simulink model "turbo_controller"  (R2025a)
settings: Solver=FixedStepAuto  StartTime=0.0  StopTime=inf  FixedStep=0.001  RelTol=1e-3
PostLoadFcn:
  | % 自动定位同目录CubeMX文件；不需要外部初始化脚本。
  | codertarget.data.setParameterValue('turbo_controller','STM32CubeMX.ProjectFile',fullfile(fileparts(get_param('turbo_controller','FileName')),'turbo_f407.ioc'));
InitFcn:
  | % 中文说明：按原控制器字段与类型创建三组接口总线；控制参数已内嵌。
  | tc_names=["EValve_Cycle" "EValve_Open" "Eblast_Cycle" "Eblast_Open" "Motor_Cycle" "Motor_Open" "EValve_Enable" "Eblast_Enable" "Motor_Enable" "SWO_Firework" "SWO_BleedAir" "EngineState" "Flag_ECUReset_Clear" "Flag_ECUReset_Save" "Flag_Reset_Enable" "Accelerator" "Nc_dem" "Nc"]; tc_types=["uint16" "uint16" "uint16" "uint16" "uint16" "uint16" "uint8" "uint8" "uint8" "uint8" "uint8" "uint8" "uint8" "uint8" "uint8" "single" "single" "single"];
  | for tc_k=1:numel(tc_names)
  |  tc_e(tc_k)=Simulink.BusElement; tc_e(tc_k).Name=char(tc_names(tc_k)); tc_e(tc_k).DataType=char(tc_types(tc_k));
  | end
  | EngineControl_Out=Simulink.Bus; EngineControl_Out.DataScope='Exported'; EngineControl_Out.Elements=tc_e;
  | clear tc_e tc_names tc_types tc_k
  | tc_names=["savedata1" "savedata2" "savedata3" "savedata4" "savedata5" "savedata6" "savedata7" "savedata8" "savedata9" "savedata10" "savedata11" "savedata12" "savedata13" "savedata14" "savedata15" "savedata16" "savedata17" "savedata18" "savedata19" "savedata20" "savedata21" "savedata22" "savedata23" "savedata24" "savedata25"]; tc_types=["single" "single" "single" "single" "single" "single" "single" "single" "single" "single" "single" "single" "single" "single" "single" "single" "single" "single" "single" "single" "single" "single" "single" "single" "single"];
  | for tc_k=1:numel(tc_names)
  |  tc_e(tc_k)=Simulink.BusElement; tc_e(tc_k).Name=char(tc_names(tc_k)); tc_e(tc_k).DataType=char(tc_types(tc_k));
  | end
  | SaveData_Out=Simulink.Bus; SaveData_Out.DataScope='Exported'; SaveData_Out.Elements=tc_e;
  | clear tc_e tc_names tc_types tc_k
  | tc_names=["senddata1" "senddata2" "senddata3" "senddata4" "senddata5" "senddata6" "senddata7" "senddata8" "senddata9" "senddata10" "senddata11" "senddata12" "senddata13" "senddata14" "senddata15" "senddata16" "senddata17" "senddata18" "senddata19" "senddata20" "senddata21" "senddata22" "senddata23" "senddata24" "senddata25" "senddata26" "senddata27" "senddata28" "senddata29"]; tc_types=["uint8" "uint8" "uint8" "uint8" "uint8" "uint8" "uint8" "uint8" "uint8" "uint8" "uint8" "uint8" "uint8" "uint8" "uint8" "uint8" "uint8" "uint8" "uint8" "uint8" "uint8" "uint8" "uint8" "uint8" "uint8" "uint8" "uint8" "uint8" "uint8"];
  | for tc_k=1:numel(tc_names)
  |  tc_e(tc_k)=Simulink.BusElement; tc_e(tc_k).Name=char(tc_names(tc_k)); tc_e(tc_k).DataType=char(tc_types(tc_k));
  | end
  | SendData_Out=Simulink.Bus; SendData_Out.DataScope='Exported'; SendData_Out.Elements=tc_e;
  | clear tc_e tc_names tc_types tc_k
  | 
  | % 以下为接口中文说明；只设置描述，不改变数值或数据类型。
  | EngineControl_Out.Description='执行控制输出（阀、电机、点火、状态及复位请求）';
  | tc_cn=["EValve_Cycle（主油阀周期计数（每计数2毫秒））" "EValve_Open（主油阀开通计数（每计数2毫秒））" "Eblast_Cycle（副油阀周期计数（每计数2毫秒））" "Eblast_Open（副油阀开通计数（每计数2毫秒））" "Motor_Cycle（起动电机周期计数）" "Motor_Open（起动电机开通计数）" "EValve_Enable（主油阀驱动使能）" "Eblast_Enable（副油阀驱动使能）" "Motor_Enable（起动电机使能）" "SWO_Firework（点火器使能（1开））" "SWO_BleedAir（引气阀使能（1开））" "EngineState（发动机状态）" "Flag_ECUReset_Clear（清除复位恢复状态请求）" "Flag_ECUReset_Save（保存复位恢复数据请求）" "Flag_Reset_Enable（处理器软件复位请求）" "Accelerator（油门／油泵给定控制量）" "Nc_dem（控制目标转速）" "Nc（发动机反馈转速（转每分））"];
  | tc_elements=EngineControl_Out.Elements;
  | for tc_k=1:numel(tc_cn)
  |  tc_elements(tc_k).Description=char(tc_cn(tc_k));
  | end
  | EngineControl_Out.Elements=tc_elements;
  | clear tc_cn tc_elements tc_k
  | SaveData_Out.Description='25项运行记录；字段含义按当前模型数据来源解释';
  | tc_cn=["savedata1（指令回显记录）" "savedata2（入口总温记录（℃））" "savedata3（电源电压记录）" "savedata4（排气温度记录（℃））" "savedata5（标定燃油压力记录）" "savedata6（副油阀占空比记录（％））" "savedata7（主油阀占空比记录（％））" "savedata8（温度修正转速记录）" "savedata9（开关输出及反馈位域）" "savedata10（物理转速记录）" "savedata11（油泵目标给定原始值）" "savedata12（起动电机占空比记录（％））" "savedata13（发动机状态码记录）" "savedata14（故障告警位域记录）" "savedata15（模型记录帧序号）" "savedata16（处理器温度记录（℃））" "savedata17（装订转速记录（沿用旧电源字段名））" "savedata18（导航高度记录）" "savedata19（飞行空速记录）" "savedata20（主阀旧记录位（恒零保留））" "savedata21（第21项保留记录（恒零））" "savedata22（保留记录项22）" "savedata23（保留记录项23）" "savedata24（保留记录项24）" "savedata25（保留记录项25）"];
  | tc_elements=SaveData_Out.Elements;
  | for tc_k=1:numel(tc_cn)
  |  tc_elements(tc_k).Description=char(tc_cn(tc_k));
  | end
  | SaveData_Out.Elements=tc_elements;
  | clear tc_cn tc_elements tc_k
  | SendData_Out.Description='29字段回传及外设命令接口；板端上位机帧只取第3至27字段';
  | tc_cn=["senddata1（回传发送允许标志（不直接上线路））" "senddata2（回传载荷长度25字节）" "senddata3（回传指令回显字节）" "senddata4（总温编码字节（℃＋80））" "senddata5（电源电压编码字节）" "senddata6（排温编码高字节）" "senddata7（排温编码低字节）" "senddata8（燃油压力编码高字节）" "senddata9（燃油压力编码低字节）" "senddata10（副油阀占空比字节（％））" "senddata11（主油阀占空比字节（％））" "senddata12（修正转速编码高字节）" "senddata13（修正转速编码低字节）" "senddata14（驱动及反馈状态位域）" "senddata15（物理转速编码高字节）" "senddata16（物理转速编码低字节）" "senddata17（油泵目标给定高字节（串口二使用））" "senddata18（油泵目标给定低字节（串口二使用））" "senddata19（起动电机占空比命令（串口一使用））" "senddata20（发动机状态码字节）" "senddata21（故障告警位域字节）" "senddata22（帧序号占位（板端另行填写））" "senddata23（处理器温度编码（℃＋50））" "senddata24（控制目标转速编码高字节）" "senddata25（控制目标转速编码低字节）" "senddata26（占位字节（板端改填实测泵速高字节））" "senddata27（占位字节（板端改填实测泵速低字节））" "senddata28（装订转速高字节（本板未发送））" "senddata29（装订转速低字节（本板未发送））"];
  | tc_elements=SendData_Out.Elements;
  | for tc_k=1:numel(tc_cn)
  |  tc_elements(tc_k).Description=char(tc_cn(tc_k));
  | end
  | SendData_Out.Elements=tc_elements;
  | clear tc_cn tc_elements tc_k
  | 
  | 
  | % FRAM模块化事务：接口类型和上电初始状态，随模型保存，无外部初始化文件。
  | clear FM_elements
  | FM_elements(1)=Simulink.BusElement;FM_elements(1).Name='phase';FM_elements(1).DataType='uint8';FM_elements(1).Dimensions=[1 1];FM_elements(1).Description='phase（当前事务阶段）';
  | FM_elements(2)=Simulink.BusElement;FM_elements(2).Name='a';FM_elements(2).DataType='uint8';FM_elements(2).Dimensions=[64 1];FM_elements(2).Description='a（启动时缓存的首区64字节）';
  | FM_elements(3)=Simulink.BusElement;FM_elements(3).Name='active';FM_elements(3).DataType='uint16';FM_elements(3).Dimensions=[1 1];FM_elements(3).Description='active（当前有效记录区地址）';
  | FM_elements(4)=Simulink.BusElement;FM_elements(4).Name='generation';FM_elements(4).DataType='uint32';FM_elements(4).Dimensions=[1 1];FM_elements(4).Description='generation（当前有效记录代号）';
  | FM_elements(5)=Simulink.BusElement;FM_elements(5).Name='record';FM_elements(5).DataType='uint8';FM_elements(5).Dimensions=[64 1];FM_elements(5).Description='record（本次冻结的待写记录）';
  | FM_elements(6)=Simulink.BusElement;FM_elements(6).Name='addr';FM_elements(6).DataType='uint16';FM_elements(6).Dimensions=[1 1];FM_elements(6).Description='addr（本次备用写入地址）';
  | FM_elements(7)=Simulink.BusElement;FM_elements(7).Name='lastSave';FM_elements(7).DataType='single';FM_elements(7).Dimensions=[1 1];FM_elements(7).Description='lastSave（上次开始保存的秒数）';
  | FM_elements(8)=Simulink.BusElement;FM_elements(8).Name='lastState';FM_elements(8).DataType='uint8';FM_elements(8).Dimensions=[1 1];FM_elements(8).Description='lastState（上次保存时的发动机状态）';
  | FM_elements(9)=Simulink.BusElement;FM_elements(9).Name='boot';FM_elements(9).DataType='boolean';FM_elements(9).Dimensions=[1 1];FM_elements(9).Description='boot（启动记录是否允许恢复）';
  | FM_elements(10)=Simulink.BusElement;FM_elements(10).Name='consumed';FM_elements(10).DataType='boolean';FM_elements(10).Dimensions=[1 1];FM_elements(10).Description='consumed（本次启动恢复通知是否已发送）';
  | FM_elements(11)=Simulink.BusElement;FM_elements(11).Name='payload';FM_elements(11).DataType='uint8';FM_elements(11).Dimensions=[20 1];FM_elements(11).Description='payload（当前20字节恢复内容）';
  | ... (+35 lines)
model workspace (MAT data in the model file):
  CRC16_Table_Reference = [0 4129 8258 12387 16516 20645 24774 28903 33032 37161 41290 45419 ... (256 elements, 256x1)]
  PE_Kaer = [0.15402 0.15402 0.12264 0.10076 0.09481 0.07601 0.07111 0.0569 0.05198 0.04926 0.05308 0.04325 ... (13 elements, 1x13)]
  PE_Nr = [21.2982 61.4260372 67.7475458 72.7394382 76.845934 80.6988798 83.8449282 86.6491912 88.9382406 89.178606 91.1938214 93.4068058 ... (13 elements, 1x13)]
  PE_Pump_Translate = 33.5999984741
  PE_RotaSpeed_Translate = 860
  PE_Taer = [0.4939154 0.4939154 0.40780982 0.34066978 0.31622756 0.30405716 0.34300244 0.26785022 0.37393554 0.23914836 0.44563948 0.31044662 ... (13 elements, 1x13)]
  PF_ACCFULLRANGE = 3360
  PF_Flag_ECUReset = 0
  PF_Flag_rx_suc = 1
  PF_Gear_Info = [40000; 45000; 50000; 55000; 57000; 59000; 60000; 61000; 61000; 61000; 61000; 61000]
  PF_K_TiaoJie = 1
  PF_Kpu = 10
  PF_MySet_Rxdata = [0 0 0 0 0 0 0 0 0 0 0 0 ... (50 elements, 50x1)]
  PF_MyUsart1_Rxdata = [0 0 0 0 0 0 0 0 0 0 0 0 ... (50 elements, 50x1)]
  PF_MyUsart2_Rxdata = [0 0 0 0 0 0 0 0 0 0 0 0 ... (50 elements, 50x1)]
  PF_Reset_Information = [0 0 0 0 0 0 0 0 0 0 0 0 ... (20 elements, 20x1)]
  PF_Sensor_X1_T4 = [0 4095]
  PF_Sensor_X2_T4 = [0 1.66666698456]
  PF_Sensor_X3_T4 = [0 504 999 1497 2010 2529 3051 3568 4076 4571 4959]
  PF_Sensor_X_P2 = [0.5 3]
  PF_Sensor_X_Poil = [0.5 3]
  PF_Sensor_X_T1t = [-50 300]
  PF_Sensor_X_Vpower = [0 3]
  PF_Sensor_X_Vpump = [0 3]
  PF_Sensor_Y1_T4 = [0 3]
  PF_Sensor_Y2_T4 = [0 5000]
  PF_Sensor_Y3_T4 = [0 100 200 300 400 500 600 700 800 900 980]
  PF_Sensor_Y_P2 = [0 1000]
  PF_Sensor_Y_Poil = [0 1000]
  PF_Sensor_Y_T1t = [-50 300]
  PF_Sensor_Y_Vpower = [0 33]
  PF_Sensor_Y_Vpump = [0 33]
  PG_CtrlMode_CloseLoop : mpt.Parameter (value not decoded)
  PG_CtrlMode_ManualAcc : mpt.Parameter (value not decoded)
  PG_CtrlMode_Origin : mpt.Parameter (value not decoded)
  PG_CtrlMode_Start : mpt.Parameter (value not decoded)
  PG_CtrlMode_Stop : mpt.Parameter (value not decoded)
  PG_ES_Clp : mpt.Parameter (value not decoded)
  PG_ES_EngStart : mpt.Parameter (value not decoded)
  PG_ES_Manual : mpt.Parameter (value not decoded)
  PG_ES_Origin : mpt.Parameter (value not decoded)
  PG_ES_Stop : mpt.Parameter (value not decoded)
  PG_Instr_BleedAirSet : mpt.Parameter (value not decoded)
  PG_Instr_CloseLoop : mpt.Parameter (value not decoded)
  PG_Instr_ECUReSet : mpt.Parameter (value not decoded)
  PG_Instr_EValveSet : mpt.Parameter (value not decoded)
  PG_Instr_EblastSet : mpt.Parameter (value not decoded)
  PG_Instr_Erase : mpt.Parameter (value not decoded)
  PG_Instr_FireWorkSet : mpt.Parameter (value not decoded)
  PG_Instr_ManualPlus : mpt.Parameter (value not decoded)
  PG_Instr_ManualrReduce : mpt.Parameter (value not decoded)
  PG_Instr_MotorSet : mpt.Parameter (value not decoded)
  PG_Instr_OilSet : mpt.Parameter (value not decoded)
  PG_Instr_SelfCheck : mpt.Parameter (value not decoded)
  PG_Instr_Start : mpt.Parameter (value not decoded)
  PG_Instr_Stop : mpt.Parameter (value not decoded)
  PG_Instr_StopZero : Simulink.Parameter (value not decoded)
  PG_Location_Air : Simulink.Parameter (value not decoded)
  PG_Location_Gnd : Simulink.Parameter (value not decoded)
  PG_ServoCtrlMode_CloseLoop : Simulink.Parameter (value not decoded)
  PG_ServoCtrlMode_CloseLoopMax : Simulink.Parameter (value not decoded)
  PG_ServoCtrlMode_CloseLoopMin : Simulink.Parameter (value not decoded)
  PG_ServoCtrlMode_ManualAcc : Simulink.Parameter (value not decoded)
  PG_ServoCtrlMode_ManualAccMax : Simulink.Parameter (value not decoded)
  PG_ServoCtrlMode_ManualAccMin : Simulink.Parameter (value not decoded)
  PG_SpeedDot_Permit : Simulink.Parameter (value not decoded)
  PL_EngineModel_Actuator = [0 10 100]
  PL_EngineModel_EngineStar_Press_P2 = [1013 1098.4 1099.144828 1099.931034 1103.613793 1162.662069 1143.793103 1131.006897 1123.186207 1117.6 1114 1111.806897 ... (127 elements, 1x127)]
  PL_EngineModel_EngineStar_RotaSpeed = [200 2000 9584 9660 10220 10240 10260 10288 10308 10368 10380 10408 ... (127 elements, 1x127)]
  PL_EngineModel_EngineStar_Temp_Exhaust = [128 129 129.1 130 131 131.1 132 133 134 134.1 135 135.1 ... (127 elements, 1x127)]
  PL_EngineModel_EngineStar_Time = [0.05 0.1 0.15 0.2 0.25 0.3 0.35 0.4 0.45 0.5 0.55 0.6 ... (127 elements, 1x127)]
  PL_EngineModel_IdleAbove_Nr = [0 21.2982 61.4260372 67.7475458 72.7394382 76.845934 80.6988798 83.8449282 86.6491912 88.9382406 89.178606 91.1938214 ... (14 elements, 1x14)]
  PL_EngineModel_IdleAbove_P2r = [0.986923266716 1.57907722675 1.81593881076 1.99358499877 2.23044658278 2.43770046879 2.65482358747 2.84233900814 3.03972366149 3.18776215149 3.25684678016 3.3950160375 ... (14 elements, 1x14)]
  PL_EngineModel_IdleAbove_Tempr = [0.0536001429337 1.07200285867 1.63301768805 1.63659103091 1.66875111667 1.72592460247 1.77595140254 1.86171163123 1.95461854565 2.03323208862 2.03323208862 2.13685903162 ... (14 elements, 1x14)]
  PL_EngineModel_IdleAbove_Ter = [0.42434128 0.42434128 0.42434128 0.30669408 0.23570008 0.22150128 0.1997974 0.23803274 0.16115638 0.24279948 0.13600422 0.31308354 ... (14 elements, 1x14)]
  PL_EngineModel_IdleAbove_Wfr = [0 10.142 23.8337 27.8905 31.9473 36.0041 40.0609 44.1177 48.1745 52.2313 52.7384 56.7952 ... (14 elements, 1x14)]
  PL_EngineModel_Press_P2 = [400 400 400 400 400 400 400 400 400 400]
  PL_EngineModel_Rotaspeed = [0 20000 96400]
  PL_EngineModel_Temp_Exhaust = [500 500 500 500 500 500 500 500 500 500]
  PL_Kaer = [0.1 0.1 0.1 0.1 0.1 0.1]
  PL_Nr = [50 60 70 80 90 100]
  PL_Taer = [0.1 0.1 0.1 0.1 0.1 0.1]
  Sig : Simulink.Signal (value not decoded)
  Ts_ms : Simulink.Parameter (value not decoded)
  false : Simulink.Parameter (value not decoded)
  true : Simulink.Parameter (value not decoded)
symbols that are objects in the model workspace (value not decoded): PG_CtrlMode_CloseLoop, PG_CtrlMode_ManualAcc, PG_CtrlMode_Origin, PG_CtrlMode_Start, PG_CtrlMode_Stop, PG_ES_Clp, PG_ES_EngStart, PG_ES_Manual, PG_ES_Origin, PG_ES_Stop, PG_Instr_BleedAirSet, PG_Instr_CloseLoop, PG_Instr_EblastSet, PG_Instr_ECUReSet, PG_Instr_Erase, PG_Instr_EValveSet, PG_Instr_FireWorkSet, PG_Instr_ManualPlus, PG_Instr_ManualrReduce, PG_Instr_MotorSet, PG_Instr_OilSet, PG_Instr_SelfCheck, PG_Instr_Start, PG_Instr_Stop, PG_Instr_StopZero, PG_ServoCtrlMode_CloseLoop, PG_ServoCtrlMode_CloseLoopMax, PG_ServoCtrlMode_CloseLoopMin, PG_ServoCtrlMode_ManualAcc, PG_ServoCtrlMode_ManualAccMax, PG_ServoCtrlMode_ManualAccMin, Ts_ms
libraries: simulink x97, stm32blockslib x10, stm32f4xxblockslib x8
(part 9 of 26)

== system turbo_controller/CLM/Start ==
  note: 普通起动：先记住起动前状态，再按阶段控制供油与电机
      |
      | 进入Start分支时，先保持起动前排温、油压；当前真正送入起动图的是油压参考，排温参考输出接终
      | 止端。参数支路根据滤波油压及历史参数准备初始电机开度、供油曲线和时间参数。
      |
      | Start_OpenLoop随后按A～F推进：准备、拖转、建立油压与供油、继续加速、退出起动电机、转入闭环
      | 。各阶段会同时修改油泵给定、主副油阀、电机和点火许可，并检查转速、油压与超时。
      |
      | 本系统只保留普通起动。阶段完成或异常的标志送回发动机状态管理，驱动量则经过统一输出管理后执
      | 行；内部某个阶段标志不是硬件执行成功的回执。
  note: DaYu5000
      | DaYu5000：只判断一个条件
      |
      | 把输入与5000比较，使用关系“>=”。成立输出1，不成立输出0；输出是判断标志，不是把输入缩放成
      | 该常数。
      |
      | 比较门限用于父级的分支条件，没有滤波、延时确认或锁存。例如输入恰好等于门限时，“>=、<=、==
      | ”成立，“>、<”不成立。是否需要持续确认或同时满足其他条件，由父级连线决定。
  S_SPM : Inport
      settings: AttributesFormatString=S_SPM（通信及传感器信息总线）
  S_ServoOut_Last : Inport  Port=2
      settings: AttributesFormatString=S_ServoOut_Last（伺服输出上一周期）
  S_Origin_T4 : Inport  Port=3
      settings: AttributesFormatString=S_Origin_T4（起动前保存的排温初值）
  S_Origin_POil : Inport  Port=4
      settings: AttributesFormatString=S_Origin_POil（起动前保存的燃油压力初值）
  Action Port : ActionPort  InitializeStates=reset  ActionPortLabel=case [ 1 ]:
      settings: AttributesFormatString=Action Port（动作端口）
  Bus Creator : BusCreator  Inputs=14
      settings: AttributesFormatString=Bus Creator（总线创建器）
  Bus Selector : BusSelector  OutputSignals=Sensor（传感器信息总线）.T4_Filter（滤波后排气温度）,Sensor（传感器信息总线）.Nc_Filter（滤波后转速）,Sensor（传感器信息总线）.POil_Filter（滤波后燃油压力）
      settings: AttributesFormatString=Bus Selector（总线选择器）
  Bus Selector2 : BusSelector  OutputSignals=m1（中间变量一）,m2（中间变量二）,m3（中间变量三）,m4（中间变量四）,n1（中间变量五）,n2（中间变量六）
      settings: AttributesFormatString=Bus Selector2（总线选择器2）
  Bus Selector3 : BusSelector  OutputSignals=m1（中间变量一）,m2（中间变量二）,m3（中间变量三）,m4（中间变量四）,n1（中间变量五）,n2（中间变量六）
      settings: AttributesFormatString=Bus Selector3（总线选择器3）
  Constant5 : Constant  Value=5000  OutDataTypeStr=single
      settings: AttributesFormatString=Constant5（常量5）
  Constant6 : Constant  Value=0  OutDataTypeStr=single
      settings: AttributesFormatString=Constant6（常量6）
  DaYu5000 : simulink/Logic and Bit Operations/Compare To Constant  Description=|  relop=>=  const=5000  OutDataTypeStr=boolean
      | DaYu5000：只判断一个条件
      | 
      | 把输入与5000比较，使用关系“>=”。成立输出1，不成立输出0；输出是判断标志，不是把输入缩放成该常数。
      | 
      | 比较门限用于父级的分支条件，没有滤波、延时确认或锁存。例如输入恰好等于门限时，“>=、<=、==”成立，“>、<”不成立。是否需要持续确认或同时满足其他条件，由父级连线决定。
      settings: AttributesFormatString=DaYu5000（大于五千）
  HoldFirst : Subsystem  Description=|
      | 保存进入起动时的排温和油压参考
      | 
      | 起动前的T4、油压会在进入本分支时被锁住。Hold图提供首次运行标志，外面的开关和延迟负责保存对应的传感器数值；不是Hold图自己保存两路模拟量。
      | 
      | 起动期间，即便当前排温或油压改变，参考值也保持进入时的水平。后面的起动图用“当前油压-起动前油压”判断压力是否建立。排温参考输出当前接Unused_OriginT4终止端，并未送入起动图；图内T4_01则在到达1000 rpm阶段另取当时排温。不能因为这里保持了两路，就认为两路都被采用。
      settings: AttributesFormatString=HoldFirst（保持首次）
  PG_CtrlMode_Start : Constant  Value=PG_CtrlMode_Start  OutDataTypeStr=uint8  SampleTime=-1
      settings: AttributesFormatString=PG_CtrlMode_Start（起动）
  PG_CtrlMode_Start3 : Constant  RequirementInfo={} %GIDa_444c69f1_f02a_4ad8_a0e8_71029ce8eb11  Value=Ts_ms  SampleTime=-1
      settings: AttributesFormatString=PG_CtrlMode_Start3（起动3）
  Range : Stateflow chart  Description=|  TreatAsAtomicUnit=on
      | 本实例把普通起动图产生的Accelerator限制在0～5000，输出为起动泵控制编码。图内算出的曲线即使大于5000也会在此截住。
      | 
      | 把一个数限制在允许范围内
      | 
      | 输入包括待处理值、允许下限和允许上限。先比较是否越过上限，越过就输出上限；未超过上限时再检查下限，小于下限就输出下限；落在范围内则原样通过。恰好等于边界的值也保留。
      | 
      | 计算式：输出 = min(max(输入，下限)，上限)。
      | 例如下限为0、上限为100时，输入120输出100，输入-5输出0，输入60输出60。这里不做平均、不计算变化速度，也不记住上一拍；它只防止当前数值越界。具体边界由父子系统连入，不能把此处的输出一律理解为百分比。
      settings: AttributesFormatString=Range（限幅或范围）
  Signal Conversion : SignalConversion  OverrideOpt=off
      settings: AttributesFormatString=Signal Conversion（信号转换）
  StartFault_Default : Constant  Description=原图该输出从未赋值，保持初始 false；显式常量保留现有起动总线字段。  Value=false  OutDataTypeStr=boolean
  Start_OpenLoop : Stateflow chart  Description=|  TreatAsAtomicUnit=on  RTWFcnName=Timmer  RTWFileName=MCM_Timmer
      | 普通起动的六阶段顺序控制
      | 
      | A准备：等待约1 s，记录并限制起动前油压参考，设置阀门周期、开启主副油路及电机使能。
      | B拖转：转速达到1000后进入C，开启点火并给出起动供油；约6 s仍未达到要求时走异常退出。
      | C建立油路：经过约3 s、油压相对基准上升50或已有进入标志时，调整主油阀与泵给定；按t、T参数和转速条件逐渐提高电机开通，达到100进入D。
      | D继续加速：转速超过参数n1进入E；超过约6 s未满足条件时撤销点火、清供油并设置异常阶段码。
      | E按转速供油：泵给定在(n1,m1)、(n2,m2)间按直线计算；超过13000时撤销起动电机和点火，超过20000进入F。油压持续高于700或本阶段约30 s超时也有退出分支。
      | F转闭环：转速超过28000或达到约20 s时关闭副油路；再按1 s、3 s的延迟恢复主油路和m4给定，最后申请进入闭环。
      | 
      | 转速单位rpm，T4为温度，油压阈值采用标定后的工程编码。计时统一按毫秒/Ts_ms比较；Ts_ms=20 ms时，1000 ms对应50次调用。泵曲线公式：
      | 泵给定=m1+(m2-m1)×(当前转速-n1)/(n2-n1)。
      | 
      | 这些阶段是流程标志，不是额外的AirStart或BWStart模式。电机关闭还有高转速及锁存路径，最终输出仍受父级模式和使能控制。
      settings: AttributesFormatString=Start_OpenLoop（地面起动开环时序）  RTWFcnNameOpts=Use subsystem name  RTWFileNameOpts=User specified
  Subsystem : Subsystem  Description=|
      | 为普通起动准备压力相关参数
      | 
      | 输入P来自POil_Filter（滤波燃油压力），不是环境静压或入口总压；另有和上一组供油曲线参数。初始化/计时支路控制何时继续沿用旧参数、何时采用压力查表结果，并由首次标志保存本次起动所需的初始值。
      | 
      | 滤波燃油压力按50～100的断点插值：初始电机开通NPump0由30变化到50，电机上升时间T由10变化到8，等待参数t由10变化到5。低压、高压会得到不同的起动节奏，不是直接把压力当作油泵开度。
      | 
      | 另一分支生成m1～m4和n1、n2供油曲线参数，再打成总线交给Start_OpenLoop。参数的含义是“在什么转速给多少泵编码、等待多久”，不代表实际油压已达到目标。
      settings: AttributesFormatString=Subsystem（子系统）
  Switch : Switch  Criteria=u2 ~= 0  SaturateOnIntegerOverflow=off  InputSameDT=off
      settings: AttributesFormatString=Switch（开关选择）
  Time Delay1 : UnitDelay  SampleTime=-1  HasFrameUpgradeWarning=on
      settings: AttributesFormatString=Time Delay1（时间延迟1）
  Unused_OriginT4 : Terminator
  Unused_ServoHistory : Terminator
  dth = T0-288.1 : Constant  Value=0  OutDataTypeStr=uint8  SampleTime=-1
      settings: AttributesFormatString=dth = T0-288.1（固定常量0（旧名称不参与计算））
  dth = T0-288.6 : Constant  OutDataTypeStr=uint8  SampleTime=-1
      settings: AttributesFormatString=dth = T0-288.6（固定常量1（旧名称不参与计算））
  S_CtrlMode_Start : Outport  InitialOutput=[0]
      settings: AttributesFormatString=S_CtrlMode_Start（控制模式起动）
  S_Start : Outport  Port=2
      settings: AttributesFormatString=S_Start（地面起动）
  wires:
  PG_CtrlMode_Start/1 -> S_CtrlMode_Start/1
  S_SPM/1 -> Bus Selector/1
  Start_OpenLoop/1(Accelerator) -> Range/1(In)
  Bus Creator/1 -> Signal Conversion/1
  Signal Conversion/1 -> S_Start/1
  Bus Selector/2 -> DaYu5000/1, Start_OpenLoop/2(Nc)  "<Nc_Filter（滤波后转速）>"
  Start_OpenLoop/7(Motor_Open) -> Bus Creator/7  "Motor_Open（起动电机开通计数）"
  Start_OpenLoop/6(Motor_Cycle) -> Bus Creator/6  "Motor_Cycle（起动电机周期计数）"
  Start_OpenLoop/8(EValve_Enable) -> Bus Creator/8  "EValve_Enable（主油阀使能）"
  Start_OpenLoop/5(Eblast_Open) -> Bus Creator/5  "Eblast_Open（副油阀开通计数）"
  Start_OpenLoop/9(Eblast_Enable) -> Bus Creator/9  "Eblast_Enable（副油阀使能）"
  Start_OpenLoop/4(Eblast_Cycle) -> Bus Creator/4  "Eblast_Cycle（副油阀周期计数）"
  Start_OpenLoop/10(Motor_Enable) -> Bus Creator/10  "Motor_Enable（起动电机使能）"
  Start_OpenLoop/3(EValve_Open) -> Bus Creator/3  "EValve_Open（主油阀开通计数）"
  Start_OpenLoop/11(SWO_Firework) -> Bus Creator/11  "SWO_Firework（点火器使能）"
  Start_OpenLoop/2(EValve_Cycle) -> Bus Creator/2  "EValve_Cycle（主油阀周期计数）"
  Start_OpenLoop/12(Flag_EngineState) -> Bus Creator/12  "Flag_RunState（运行状态标志）"
  S_Origin_T4/1 -> HoldFirst/1(S_Origin_T4)
  Switch/1 -> Bus Creator/14  "SWO_BleedAir（引气阀使能）"
  Bus Selector/1 -> Start_OpenLoop/1(T4)  "<T4_Filter（滤波后排气温度）>"
  PG_CtrlMode_Start3/1 -> Start_OpenLoop/13(Ts_ms)
  S_Origin_POil/1 -> HoldFirst/2(S_Origin_POil)
  HoldFirst/2(S_Origin_POil_1) -> Start_OpenLoop/14(Origin_POil)
  Bus Selector/3 -> Subsystem/1(P), Start_OpenLoop/3(POil)  "<POil_Filter（滤波后燃油压力）>"
  Constant6/1 -> Range/3(Min)
  Constant5/1 -> Range/2(Max)
  Range/1(Out) -> Bus Creator/1  "Start_Accelerator（地面起动油泵给定）"
  Time Delay1/1 -> Bus Selector2/1
  Bus Selector2/1 -> Subsystem/2(m1_last)  "<m1（中间变量一）>"
  Bus Selector2/2 -> Subsystem/3(m2_last)  "<m2（中间变量二）>"
  Bus Selector2/3 -> Subsystem/4(m3_last)  "<m3（中间变量三）>"
  Bus Selector2/4 -> Subsystem/5(m4_last)  "<m4（中间变量四）>"
  Subsystem/2(m) -> Time Delay1/1, Bus Selector3/1
  Bus Selector3/1 -> Start_OpenLoop/5(m1)  "<m1（中间变量一）>"
  Bus Selector3/2 -> Start_OpenLoop/6(m2)  "<m2（中间变量二）>"
  Bus Selector3/3 -> Start_OpenLoop/7(m3)  "<m3（中间变量三）>"
  Bus Selector3/4 -> Start_OpenLoop/8(m4)  "<m4（中间变量四）>"
  Subsystem/1(NPump0) -> Start_OpenLoop/4(NPump0)
  Subsystem/3(T) -> Start_OpenLoop/11(T)
  Bus Selector2/5 -> Subsystem/6(n1_last1)  "<n1（中间变量五）>"
  Bus Selector2/6 -> Subsystem/7(n2_last2)  "<n2（中间变量六）>"
  Bus Selector3/5 -> Start_OpenLoop/9(n1)  "<n1（中间变量五）>"
  Bus Selector3/6 -> Start_OpenLoop/10(n2)  "<n2（中间变量六）>"
  Subsystem/4(t) -> Start_OpenLoop/12(t)
  dth = T0-288.1/1 -> Switch/3
  dth = T0-288.6/1 -> Switch/1
  DaYu5000/1 -> Switch/2
  StartFault_Default/1 -> Bus Creator/13  "Flag_StartFault（起动故障标志）"
  HoldFirst/1(S_Origin_T4_0) -> Unused_OriginT4/1
  S_ServoOut_Last/1 -> Unused_ServoHistory/1

== system turbo_controller/CLM/Stop ==
  note: 【本页库子系统中文说明】TingCheZhiLing1
      | 一、它做什么？
      | 这是“过不过这条线”的判断器。将输入与阈值 PG_Instr_StopZero 作 == 比较，关
      | 系成立输出真（1），否则输出假（0）。例如>=包含恰好等于，>则不包含。它只给出
      | 判断标志，不会自行限幅、报警、切换状态或操作阀门；后续逻辑决定如何使用。名称
      | 可能只是用途提示，实际判据以这里的关系和阈值为准。
      | 二、本实例当前参数
      | 比较关系：==
      | 比较阈值：PG_Instr_StopZero
      | 输出数据类型：布尔值，真或假
      | 零交叉检测：开启
      | 三、怎样继续学习？
      | 这是标准库子系统实例。中文说明放在使用它的父级页面，并同步存入本块Descriptio
      | n（模块说明）；官方库链接保留。先看本实例的输入来自哪里、输出交给谁，再结合
      | 以上参数理解作用。
  note: 停车模式：停止供油并按条件处理尾部拖转
      |
      | 停车命令进入本分支后，常规油泵给定转为停车值，Stop_Control结合命令、当前转速、排温及运行状
      | 态决定阀门和电机动作。
      |
      | StopZero用于快速完成停车路径；普通停车保留等待、关闭油路及高温低转速时的电机拖转判断。Stop
      | _Finish输出送发动机状态管理，控制数值和使能送统一输出管理。
      |
      | “停车完成”是控制逻辑的完成标志，不是由此模块直接证明轴已完全静止。实际转速仍由独立测速链
      | 路采集。
  note: TingCheZhiLing1
      | TingCheZhiLing1：只判断一个条件
      |
      | 把输入与15比较，使用关系“==”。成立输出1，不成立输出0；输出是判断标志，不是把输入缩放成该
      | 常数。
      |
      | 这里识别一种指令编码。判断成立只说明指令匹配；父级还会结合有效帧、当前模式或其他允许条件决
      | 定是否更新。实际驱动要继续经过控制与板级输出，不能把1理解为硬件执行回执。
  S_Start : Inport
      settings: AttributesFormatString=S_Start（地面起动）
  S_SPM : Inport  Port=2
      settings: AttributesFormatString=S_SPM（通信及传感器信息总线）
  Action Port : ActionPort  InitializeStates=reset  ActionPortLabel=case [ 4 ]:
      settings: AttributesFormatString=Action Port（动作端口）
  Bus Creator : BusCreator  Inputs=13
      settings: AttributesFormatString=Bus Creator（总线创建器）
  Bus Selector : BusSelector  OutputSignals=Sensor（传感器信息总线）.Nc_Filter（滤波后转速）,Sensor（传感器信息总线）.T4_Filter（滤波后排气温度）,COMM（通信信息总线）.Instr（控制指令）
      settings: AttributesFormatString=Bus Selector（总线选择器）
  Bus Selector2 : BusSelector  OutputSignals=Flag_RunState（运行状态标志）
      settings: AttributesFormatString=Bus Selector2（总线选择器2）
  Constant1 : Constant  Value=30  OutDataTypeStr=uint16  SampleTime=-1
      settings: AttributesFormatString=Constant1（常量1）
  Constant3 : Constant  Value=30  OutDataTypeStr=uint16  SampleTime=-1
      settings: AttributesFormatString=Constant3（常量3）
  Constant4 : Constant  Value=0  OutDataTypeStr=uint8  SampleTime=-1
      settings: AttributesFormatString=Constant4（常量4）
  Constant7 : Constant  Value=100  OutDataTypeStr=uint16  SampleTime=-1
      settings: AttributesFormatString=Constant7（常量7）
  Constant8 : Constant  Value=0  OutDataTypeStr=uint8  SampleTime=-1
      settings: AttributesFormatString=Constant8（常量8）
  Divide : Product  Inputs=**
      settings: AttributesFormatString=Divide（除法）
  N1r_idle6 : Constant  Value=PG_CtrlMode_Stop  OutDataTypeStr=uint8  SampleTime=-1
      settings: AttributesFormatString=N1r_idle6（一级转速归一化值慢车6）
  PG_CtrlMode_Start1 : Constant  Value=PF_ACCFULLRANGE  OutDataTypeStr=single  SampleTime=-1
      settings: AttributesFormatString=PG_CtrlMode_Start1（起动1）
  PG_CtrlMode_Start3 : Constant  Value=Ts_ms  SampleTime=-1
      settings: AttributesFormatString=PG_CtrlMode_Start3（起动3）
  Signal Conversion : SignalConversion  OverrideOpt=off
      settings: AttributesFormatString=Signal Conversion（信号转换）
  StopMotorEnable_Default : Constant  Description=原停车状态图该输出从未赋值，保持初始 uint8(0)，保留停车总线字段。  Value=uint8(0)  OutDataTypeStr=uint8
  Stop_Control : Stateflow chart  Description=|  TreatAsAtomicUnit=on  RTWFcnName=Timmer  RTWFileName=MCM_Timmer
      | 停车中的油路关闭、电机拖转和完成判断
      | 
      | 接收停车命令、排温T4、转速Nc、原运行状态及Time_ms。StopZero分支直接置停车完成并关闭电机；普通停车先按约1 s等待条件处理阀门与供油。
      | 
      | 图内对Nc≤7000、T4≥100设置了电机开通50的拖转路径，并限制拖转计时为约15 s；还存在低温、低转速和不同运行状态的提前完成路径。条件按图上的分支顺序判断，不能把所有温度与转速比较拼成一个同时成立的条件。
      | 
      | 计时门限为等待毫秒数/Time_ms，例如Time_ms=20时15 s对应750次调用。输出是电机、油阀及Stop_Finish，随后分别进入板级输出和发动机状态转换。
      settings: AttributesFormatString=Stop_Control（停车控制）  RTWFcnNameOpts=Use subsystem name  RTWFileNameOpts=User specified
  TingCheZhiLing1 : simulink/Logic and Bit Operations/Compare To Constant  Description=|  relop===  const=PG_Instr_StopZero  OutDataTypeStr=boolean
      | TingCheZhiLing1：只判断一个条件
      | 
      | 把输入与15比较，使用关系“==”。成立输出1，不成立输出0；输出是判断标志，不是把输入缩放成该常数。
      | 
      | 这里识别一种指令编码。判断成立只说明指令匹配；父级还会结合有效帧、当前模式或其他允许条件决定是否更新。实际驱动要继续经过控制与板级输出，不能把1理解为硬件执行回执。
      settings: AttributesFormatString=TingCheZhiLing1（停车指令1）
  S_CtrlMode_Stop : Outport  InitialOutput=[0]
      settings: AttributesFormatString=S_CtrlMode_Stop（控制模式停车）
  S_Stop : Outport  Port=2  OutputWhenDisabled=reset  InitialOutput=[0]
      settings: AttributesFormatString=S_Stop（停车）
  wires:
  PG_CtrlMode_Start1/1 -> Divide/1
  Constant4/1 -> Bus Creator/13  "SWO_BleedAIr（引气阀使能）"
  Stop_Control/7(StopFinish) -> Bus Creator/12  "StopFinish（停车完成标志）"
  PG_CtrlMode_Start3/1 -> Stop_Control/1(Time_ms)
  Stop_Control/1(Accelerator) -> Divide/2
  Stop_Control/6(Eblast_Enable) -> Bus Creator/9  "Eblast_Enable（副油阀使能）"
  Stop_Control/4(Motor_Open) -> Bus Creator/7  "Motor_Open（起动电机开通计数）"
  Constant8/1 -> Bus Creator/11  "SWO_Firework（点火器使能）"
  Constant7/1 -> Bus Creator/6  "Motor_Cycle（起动电机周期计数）"
  Stop_Control/5(EValve_Enable) -> Bus Creator/8  "EValve_Enable（主油阀使能）"
  Stop_Control/2(EValve_Open) -> Bus Creator/3  "EValve_Open（主油阀开通计数）"
  Constant3/1 -> Bus Creator/4  "Eblast_Cycle（副油阀周期计数）"
  Stop_Control/3(Eblast_Open) -> Bus Creator/5  "Eblast_Open（副油阀开通计数）"
  Constant1/1 -> Bus Creator/2  "EValve_Cycle（主油阀周期计数）"
  Signal Conversion/1 -> S_Stop/1
  Bus Creator/1 -> Signal Conversion/1
  Divide/1 -> Bus Creator/1  "Accelerator（油泵给定控制量）"
  N1r_idle6/1 -> S_CtrlMode_Stop/1
  S_Start/1 -> Bus Selector2/1
  Bus Selector2/1 -> Stop_Control/5(Flag_RunState)  "<Flag_RunState（运行状态标志）>"
  S_SPM/1 -> Bus Selector/1
  Bus Selector/1 -> Stop_Control/2(Nc)  "<Nc_Filter（滤波后转速）>"
  Bus Selector/2 -> Stop_Control/3(T4)  "<T4_Filter（滤波后排气温度）>"
  Bus Selector/3 -> TingCheZhiLing1/1  "<Instr（控制指令）>"
  TingCheZhiLing1/1 -> Stop_Control/4(StopZero)
  StopMotorEnable_Default/1 -> Bus Creator/10  "Motor_Enable（起动电机使能）"

== system turbo_controller/COMMRead_ISM/CMMRead ==
  note: 把已校验的上位机帧解释为命令和运行设定
      |
      | 输入是接收层保留下来的帧、接收成功标志和当前发动机模式。先由Instr_Analyse识别命令，再由Spe
      | edLoad_Analyse确定本次目标转速，同时解析高度、空速、环境温度、电压等协议字段。
      |
      | 一帧数据并不是全部都用于当前控制。命令类型决定哪些字段有效；没有新有效信息时，需要保持的设
      | 定沿用历史值。闭环目标、起动默认目标和停车目标有各自的选择路径。
      |
      | 本层负责“字节是什么意思”；校验与收帧在BoardInput内完成，实际驱动在CLM和BoardOutput完成。
      | 输出的通信电压、环境信息也不能与ADC测得的同名量混为一谈。
  S_Flag_rx_suc : Inport
      settings: AttributesFormatString=S_Flag_rx_suc（四号串口指令帧有效标志）
  S_PF_MyUsart2_Rxdata : Inport  Port=2
      settings: AttributesFormatString=S_PF_MyUsart2_Rxdata（本通道通用同步异步串行通信接口2接收数据）
  S_Flag_ECUReset_Use : Inport  Port=3
      settings: AttributesFormatString=S_Flag_ECUReset_Use（标志电子控制器复位使用）
  S_ECUReset_NcDem : Inport  Port=4
      settings: AttributesFormatString=S_ECUReset_NcDem（电子控制器复位目标转速）
  S_EngineState : Inport  Port=5
      settings: AttributesFormatString=S_EngineState（发动机状态）
  Instr_Analyse : Subsystem  Description=|
      | 识别上位机命令，并把相关数据交给对应功能
      | 
      | 从已接收帧中取出命令字段，将其与起动、停车、闭环、手动泵、阀门、电机、点火及引气等命令常量比较。带有效接收条件的选择支路更新本次指令和参数，否则保持原先设定。
      | 
      | 装订/档位另有复合编码识别，不是把整个命令字直接当作一个状态编号。输出同时包含指令结果、成功标志和需要继续解释的数据。
      | 
      | 指令描述“用户要求做什么”，EngineState描述“发动机当前处于什么模式”，两者不是一个变量。指令先进入ESM产生模式转换条件，再由CLM选择控制分支；不能因收到一条Start就认为硬件已经起动完成。
      settings: AttributesFormatString=Instr_Analyse（指令分析解析）
  SpeedLoad_Analyse : Subsystem  Description=|
      | 确定本次采用的目标转速，并记住有效目标
      | 
      | 先由Speed_Load_Cal解码候选目标，再按命令和模式选择。闭环目标只有落在40000～61000 rpm的允许范围内才走相应更新路径；有效起动命令且处于初始模式时装订40000；停车命令走0目标路径。
      | 
      | 当没有满足条件的新设定时，继续使用延迟保存的原目标。复位恢复路径可选择保存过的NcDem，但还要求恢复有效及初始模式；当前上层恢复使能固定false，这条路径不会正常投入。
      | 
      | 例如原目标50000，新闭环目标55000且条件有效时更新为55000；不满足更新条件则继续50000。这里输出的是期望值，实际转速由传感器测得，CLM再对两者差值进行控制。
      settings: AttributesFormatString=SpeedLoad_Analyse（装订转速指令解析）
  T1t_P1t_Cal : Subsystem  Description=|
      | 解释飞行环境字段，并计算进气总温、总压
      | 
      | 从通信帧提取高度、空速、温度及电压编码，按各通道比例与偏置恢复数值。有效接收时更新需要保持的高度信息；H0_T0图负责设定值和高度变化信息的保持。
      | 
      | 高度由米换成千米后送Dynamic_Cal。它先按高度得到静温、静压，再把空速造成的气流减速升温、升压计入，输出总温T1t和总压P1t。标准海平面参考压力为101.325，温度计算要用K，不能直接把摄氏度代入平方根。
      | 
      | 这里是根据上位机信息估算的环境，不是ADC总温电阻的换算。当前父级送ISM的转速修正温度仍采用288.15 K常量，不能以为此处算出的总温已经接入所有下游控制。
      settings: AttributesFormatString=T1t_P1t_Cal（入口总温入口总压计算）
  S_Rx_suc : Outport
      settings: AttributesFormatString=S_Rx_suc（接收数据成功或有效）
  S_Instr_XianShi : Outport  Port=2
      settings: AttributesFormatString=S_Instr_XianShi（指令显示显示）
  S_Instr_Out : Outport  Port=3
      settings: AttributesFormatString=S_Instr_Out（指令输出）
  S_SpeedLoad : Outport  Port=4
      settings: AttributesFormatString=S_SpeedLoad（装订转速）
  T0_calc : Outport  Port=5
      settings: AttributesFormatString=T0_calc（环境温度计算）
  T1t_calc : Outport  Port=6
      settings: AttributesFormatString=T1t_calc（入口总温计算）
  P1t_calc : Outport  Port=7
      settings: AttributesFormatString=P1t_calc（入口总压计算）
  H_GPRS : Outport  Port=8
      settings: AttributesFormatString=H_GPRS（导航高度）
  AirSpeed : Outport  Port=9
      settings: AttributesFormatString=AirSpeed（空速）
  S_COMM_Data6 : Outport  Port=10
      settings: AttributesFormatString=S_COMM_Data6（通信数据6）
  H_Load : Outport  Port=11
      settings: AttributesFormatString=H_Load（装订高度）
  V_Power : Outport  Port=12
      settings: AttributesFormatString=V_Power（电压或控制量变量电源）
  wires:
  S_PF_MyUsart2_Rxdata/1 -> [PF_MyUsart2_Rxdata]
  [PF_MyUsart2_Rxdata] -> Instr_Analyse/1(S_MyUsart2_Rxdata)
  [Rx_suc] -> Instr_Analyse/2(S_Rx_suc)
  [Rx_suc] -> S_Rx_suc/1
  S_Flag_rx_suc/1 -> [Rx_suc]
  Instr_Analyse/2(S_Instr_Out) -> S_Instr_Out/1, SpeedLoad_Analyse/1(S_Instr_Out)
  Instr_Analyse/1(S_Instr_XianShi) -> S_Instr_XianShi/1
  SpeedLoad_Analyse/1(S_SpeedLoad) -> S_SpeedLoad/1
  [PF_MyUsart2_Rxdata] -> SpeedLoad_Analyse/3(S_MyUsart2_Rxdata)
  [Rx_suc] -> SpeedLoad_Analyse/2(S_Rx_suc)
  T1t_P1t_Cal/1(S_T0_calc) -> T0_calc/1
  [PF_MyUsart2_Rxdata] -> T1t_P1t_Cal/1(S_PF_MyUsart2_Rxdata)
  T1t_P1t_Cal/2(S_T1t_calc) -> T1t_calc/1
  T1t_P1t_Cal/3(S_P1t_calc) -> P1t_calc/1
  T1t_P1t_Cal/4(S_H_GPRS) -> H_GPRS/1
  T1t_P1t_Cal/5(S_AirSpeed) -> AirSpeed/1
  [Rx_suc] -> T1t_P1t_Cal/2(S_Rx_suc)
  S_ECUReset_NcDem/1 -> SpeedLoad_Analyse/5(S_ECUReset_NcDem)
  S_Flag_ECUReset_Use/1 -> SpeedLoad_Analyse/4(S_Flag_ECUReset_Use)
  S_EngineState/1 -> SpeedLoad_Analyse/6(S_EngineState)
  Instr_Analyse/3(S_COMM_Data6) -> S_COMM_Data6/1
  T1t_P1t_Cal/6(S_H_Load) -> H_Load/1
  T1t_P1t_Cal/7(S_V_Power) -> V_Power/1

== system turbo_controller/COMMRead_ISM/ECUReset_Information_Read ==
  note: 从恢复字节中取回泵给定、目标转速和原运行模式
      |
      | 输入是FRAM恢复信息数组与有效标志。泵给定用两个字节高位在前合成，目标转速用三个字节合成；发
      | 动机模式由指定字节直接取出。
      |
      | 有效恢复不只看数组里有没有非零值，还要经过目标转速30000～89000的范围判断并与恢复标志组合。
      | 输出分别供目标选择、恢复期间泵输出及模式判断使用。
      |
      | 当前COMMRead_ISM把恢复标志接为false，尽管这些解码支路仍在，正常运行不会采用恢复记录。不要
      | 把“可以解码”解释为“复位后已经按该值恢复运行”。
  S_Flag_ECUReset : Inport
      settings: AttributesFormatString=S_Flag_ECUReset（复位恢复标志）
  S_ECUReset_Information : Inport  Port=2
      settings: AttributesFormatString=S_ECUReset_Information（铁电存储器中的复位恢复记录）
  ECUReset_Acclerator_Cal : Subsystem  Description=|
      | 把保存的两个字节还原成油泵给定
      | 
      | 按高字节在前合成：泵给定=高字节×256+低字节。例如高字节11、低字节184，恢复得到3000。
      | 
      | 这里只恢复无符号控制编码，不换算成燃油流量，不根据电压补偿，也不验证整条FRAM记录。记录校验、恢复是否允许和最终是否采用该值在事务层及父级完成。输入字段位置按恢复信息协议排列，不能随意调换高低字节。
      settings: AttributesFormatString=ECUReset_Acclerator_Cal（控制器复位油门计算）
  ECUReset_Information_EngineState : Selector  IndexMode=Zero-based  InputPortWidth=20  IndexOptions=Index vector (dialog)  Indices=[8]  OutputSizes=1
      settings: AttributesFormatString=ECUReset_Information_EngineState（控制器复位信息发动机状态）
  Flag_ECUReset_Manage : Subsystem  Description=|
      | 还原保存的目标转速，并判定可否采用
      | 
      | 从恢复信息中取出三个字节，高字节在前合成：
      | 目标rpm=高字节×65536+中字节×256+低字节。
      | 例如0、195、80合成50000。
      | 
      | 目标在30000～89000之间才满足本模块的数值范围要求，再与外部恢复有效标志组合，形成恢复使用许可。范围合法仅说明数值像一个允许的目标，不能代替FRAM记录校验；外部标志为假时仍不采用。
      | 
      | 目标输出继续送SpeedLoad_Analyse，最终还取决于当前模式和恢复选择。当前上层使能固定false，因此本模块的解码结果不会自行激活闭环。
      settings: AttributesFormatString=Flag_ECUReset_Manage（标志控制器复位管理）
  S_Flag_ECUReset_Use : Outport
      settings: AttributesFormatString=S_Flag_ECUReset_Use（标志电子控制器复位使用）
  S_ECUReset_Acclerator : Outport  Port=2
      settings: AttributesFormatString=S_ECUReset_Acclerator（电子控制器复位油门）
  S_ECUReset_NcDem : Outport  Port=3
      settings: AttributesFormatString=S_ECUReset_NcDem（电子控制器复位目标转速）
  S_ECUReset_EngineState : Outport  Port=4
      settings: AttributesFormatString=S_ECUReset_EngineState（电子控制器复位发动机状态）
  wires:
  S_ECUReset_Information/1 -> ECUReset_Information_EngineState/1, ECUReset_Acclerator_Cal/1(S_ECUReset_Information), Flag_ECUReset_Manage/1(S_ECUReset_Information)
  ECUReset_Information_EngineState/1 -> S_ECUReset_EngineState/1
  S_Flag_ECUReset/1 -> Flag_ECUReset_Manage/2(S_Flag_ECUReset)
  Flag_ECUReset_Manage/1(S_Flag_ECUReset_Process) -> S_Flag_ECUReset_Use/1
  ECUReset_Acclerator_Cal/1(S_ECUReset_Acclerator) -> S_ECUReset_Acclerator/1
  Flag_ECUReset_Manage/2(S_ECUReset_NcDem) -> S_ECUReset_NcDem/1

== system turbo_controller/COMMRead_ISM/ISM ==
  note: 把测量输入整理成控制算法能取用的Sensor总线
      |
      | 本层接收的输入并不全是同一类数据：排温、油压和芯片温度仍有原始计数；电源电压已经在BoardInp
      | ut换算成V；T0则是加80后的温度编码。先认清这一点，才能理解为什么各路处理不同。
      |
      | 排温走Calibrating_T4三级查表，再走AnalogFilter_T4，得到平滑的T4_Filter。标定后的排温还分一
      | 路到Subsystem2，以930 ℃上限生成排温超限标志；这一路标志当前没有查到下游取用。
      | 油压走Calibrating_Poil，将计数换为电压、再换为压力，然后AnalogFilter_Poil平滑，得到POil_Fi
      | lter。
      | 芯片温度走Calibrating_Tecu，先换电压，再按0.76 V和25 ℃参考关系计算Tecu。
      | 总温走Calibrating_T0，减去80并限制在-70～175 ℃；再与原位滤波转速送入HuanSuanN，计算温度修
      | 正转速。
      | 电源电压Vpower已经是V，本层直接转交，不再做独立低通滤波。
      |
      | 转速来自捕获/电机链路，不来自ADC。它一方面进入AnalogFilter_Nc作异常检查和滤波；另一方面进
      | 入Origin_Nc_Filter，形成原位转速，供总温修正使用。
      | 点火、阀门等数字反馈按字段转交。
      |
      | 最后Bus Creator3按名称把上述结果装进Sensor总线，再由父级与COMM总线合成S_SPM。总线只是打包
      | ，不再次计算数值。CLM、MAM、SaveData和SendData分别取所需字段，因此标定值、滤波值和故障标志
      | 要分开理解。
  S_T1t_calc : Inport
      settings: AttributesFormatString=S_T1t_calc（入口总温计算）
  S_T4 : Inport  Port=2
      settings: AttributesFormatString=S_T4（排温ADC采样码（未换算℃））
  S_Vpower : Inport  Port=3
      settings: AttributesFormatString=S_Vpower（板端换算电源电压）
  S_Tecu : Inport  Port=4
      settings: AttributesFormatString=S_Tecu（处理器温度ADC采样码）
  S_Nc : Inport  Port=5
      settings: AttributesFormatString=S_Nc（发动机反馈转速（转每分））
  S_SWI_Firework : Inport  Port=6
      settings: AttributesFormatString=S_SWI_Firework（点火器报警反馈（低有效））
  S_SWI_EValve : Inport  Port=7
      settings: AttributesFormatString=S_SWI_EValve（主油阀反馈（低有效））
  S_SWI_Eblast : Inport  Port=8
      settings: AttributesFormatString=S_SWI_Eblast（副油阀反馈（低有效））
  S_SWI_ValveErr : Inport  Port=9
      settings: AttributesFormatString=S_SWI_ValveErr（任一路阀报警（低有效））
  S_EngineState : Inport  Port=10
      settings: AttributesFormatString=S_EngineState（发动机状态）
  S_SWI_BleedAir : Inport  Port=11
      settings: AttributesFormatString=S_SWI_BleedAir（引气阀反馈（低有效））
  S_POil : Inport  Port=12
      settings: AttributesFormatString=S_POil（油压输入：模型需采样码／板端传电压）
  S_T0 : Inport  Port=13
      settings: AttributesFormatString=S_T0（板端总温编码（℃＋80））
  AnalogFilter_Nc : Subsystem  Description=|
      | 检查转速可信度，并形成控制转速及相对转速
      | 
      | 先按模式设置转速下限：闭环时采用10000，其他模式采用0；上限70000。GeneralFilter同时检查相邻两拍变化，突变量门限1200、恢复门限800、恢复确认参数100 ms。
      | 
      | 异常样本可能被上一有效值替代，然后进行一阶低通，得到Nc_Filter。范围故障与变化故障分别输出，供FPM决定暂时保持控制还是采用故障备份曲线。
      | 
      | 相对转速以61000 rpm为100%：百分比=当前转速×100/61000。另有按温度sqrt(288.15/T1t_calc)修正的转速及百分比。温度必须为K；当前此输入由上层接288.15 K，修正系数为1。不要与独立的ADC总温修正记录通道混淆。
      settings: AttributesFormatString=AnalogFilter_Nc（转速滤波与故障判断）
  AnalogFilter_Poil : Subsystem  Description=|
      | 对标定后的油压做一阶低通，减小采样抖动
      | 
      | 每次把本拍输入与上次滤波结果按比例相加：
      | 本拍输出=α×本拍输入+β×上次输出；
      | α=Ts/(T+Ts)，β=T/(T+Ts)。
      | 
      | 当前T=0.067 s，Ts=Ts_ms/1000=0.02 s，因此α约0.229885、β约0.770115。新输入约占23%，旧结果约占77%。例如上次输出100、本次输入200，本次滤波结果约123，随后逐步靠近200。
      | 
      | 它抑制快速波动，也会让真实变化稍有滞后；不负责把ADC计数变成物理量，也不单凭滤波判定传感器故障。输出送POil_Filter，供起动阶段比较压力建立情况并用于记录。
      settings: AttributesFormatString=AnalogFilter_Poil（燃油压力滤波）
  AnalogFilter_T4 : Subsystem  Description=|
      | 对标定后的排温做一阶低通，减小采样抖动
      | 
      | 每次把本拍输入与上次滤波结果按比例相加：
      | 本拍输出=α×本拍输入+β×上次输出；
      | α=Ts/(T+Ts)，β=T/(T+Ts)。
      | 
      | 当前T=0.067 s，Ts=Ts_ms/1000=0.02 s，因此α约0.229885、β约0.770115。新输入约占23%，旧结果约占77%。例如上次输出100、本次输入200，本次滤波结果约123，随后逐步靠近200。
      | 
      | 它抑制快速波动，也会让真实变化稍有滞后；不负责把ADC计数变成物理量，也不单凭滤波判定传感器故障。输出送T4_Filter，供起动、告警与记录。
      settings: AttributesFormatString=AnalogFilter_T4（排温滤波）
  Bus Creator3 : BusCreator  Inputs=19
      settings: AttributesFormatString=Bus Creator3（总线创建器3）
  Calibrating_Poil : Subsystem  Description=|
      | 油压计数怎样换成压力
      | 
      | 输入来自BoardInput的ADC第8项，仍是single类型的ADC计数。本模块依次经过两张线性查表，输出压力工程量，随后交给AnalogFilter_Poil平滑。
      | 
      | 第一张Bit2V表把0～4095计数映射为0～3.3 V：
      | 传感器电压 = ADC计数 × 3.3 / 4095。
      | 第二张POil_X_Y表采用0.5 V对应0、3.0 V对应1000：
      | 压力 = (传感器电压 - 0.5) / 2.5 × 1000。
      | 
      | 例如电压为1.75 V时，恰好在0.5和3.0 V中点，得到压力500。两张表超出断点时都采用端点值，所以最终量程为0～1000，而不是继续向表外延伸。
      | 
      | 这里能从参数确定量程，压力单位应与实际传感器和工程约定对应。本模块没有做滤波，也没有生成油压故障标志；这些不能从“标定”二字推断出来。下一级滤波后的POil_Filter用于原位、普通起动、记录和回传。
      settings: AttributesFormatString=Calibrating_Poil（油压采样码标定（板端单位待对齐））
  Calibrating_T0 : Subsystem  Description=|
      | 把总温编码还原成摄氏温度
      | 
      | 输入来自BoardInput/TotalTemperature。那一路已用两路ADC反算电阻并计算温度，但为了沿用接口格式，输出时额外加了80。本模块先减掉这个偏置：
      | 摄氏总温 = 输入编码 - 80。
      | 
      | 随后Range把结果限制在-70～175 ℃。例如输入105，减80后得到25 ℃；输入300，原结果220 ℃超过上限，最后输出175 ℃。限幅只是约束数值范围，不会单独输出断线或超温故障。
      | 
      | 处理后的Sensor.T0一路给SaveData和SendData记录回传，另一路给HuanSuanN，与原位滤波转速计算温度修正转速。本模块没有独立低通滤波。
      | 注意：上游无效电压差可能被替代为R=9999，最终也会走到175 ℃上限，因此175 ℃可能是限幅/替代结果。
      settings: AttributesFormatString=Calibrating_T0（总温编码减80并限幅）
  Calibrating_T4 : Subsystem  Description=|
      | 排温计数怎样经过三级标定
      | 
      | 输入来自ADC第4项，BoardInput仅完成single转换。当前计数依次经过三张表，而不是直接乘一个温度系数。
      | 
      | 第一张T4_X1_Y1把0～4095计数映射到0～3 V，等价于V=计数×3/4095。
      | 第二张T4_X2_Y2把0～约1.666667 V映射到0～5000的传感器标定中间量；这仍不是摄氏温度。
      | 第三张T4_X3_Y3根据非线性标定表，把中间量换成排温。例如中间量504对应100 ℃、999对应200 ℃、2529对应500 ℃、4959对应980 ℃。504是第三级表的输入，不是原ADC计数。
      | 
      | 每张表在相邻断点间线性插值：输出=左端输出+(右端输出-左端输出)×当前位置比例。若输入超出表范围，采用该表端点值。这样分别表达电路比例和传感器非线性。
      | 
      | 输出排温分两路：一路送AnalogFilter_T4作0.067 s一阶滤波，供起动、停车、冷吹和850 ℃告警；另一路在滤波前送Subsystem2作930 ℃超限判断。这里没有直接驱动阀门，也没有直接发停车命令。
      settings: AttributesFormatString=Calibrating_T4（排温采样码分段标定）
  Calibrating_Tecu : Subsystem  Description=|
      | 芯片内部温度计数怎样换成摄氏温度
      | 
      | 输入是ADC数组第3项，对应STM32内部温度传感器。它不是排气温度，也不是环境总温。
      | 
      | 先用Bit2V表把0～4095计数映射到0～3.0 V，得到传感器电压V。随后按当前模型的参考点和斜率计算：
      | Tecu = (V - 0.76) × 400 + 25，单位℃。
      | 
      | 0.76 V对应25 ℃；电压比参考值增加0.01 V时，按本公式温度增加4 ℃。这里的400是当前采用的摄氏度/伏特比例，实际标定是否适合硬件要以传感器参数为依据。
      | 
      | 输出组成Sensor.Tecu，主要交给SaveData记录和SendData回传。当前没有查到独立的控制器过温停车分支，也没有在这里低通滤波。SendData会加50、限制到0～255，再变成字节；例如25 ℃回传编码约为75。
      settings: AttributesFormatString=Calibrating_Tecu（处理器温度采样码标定）
  Data Type Conversion2 : DataTypeConversion  OutDataTypeStr=single  SaturateOnIntegerOverflow=off  RndMeth=Floor
      settings: AttributesFormatString=Data Type Conversion2（数据类型转换2）
  HuanSuanN : Subsystem  Description=|
      | 用总温修正原位转速
      | 
      | 实际转速会随环境温度产生不同的工作含义。这里接收Origin_Nc_Filter的原位滤波转速N，以及Calibrating_T0的摄氏总温T0，计算一个按参考温度归一化的转速。
      | 
      | 先把摄氏温度变成绝对温度：Tk=273.15+T0，单位K。
      | 再计算温度比例的平方根，并乘实际转速：
      | 修正转速 = N × sqrt(288.15 / Tk)。
      | 最后Range把结果限制到0～75000。
      | 
      | 例如T0=15 ℃时Tk=288.15 K，比例为1，修正前后相同；温度更低时比例大于1，温度更高时比例小于1。输入N与输出采用同一转速单位。
      | 
      | 输出名为HuanSuanZhuanSu。当前它被SaveData和SendData取出，用于记录与回传，没有查到直接作为闭环反馈使用。闭环用的Nc_Filter是另一条滤波转速，不要把两者混成一个变量。
      settings: AttributesFormatString=HuanSuanN（按入口总温修正转速）
  Origin_Nc_Filter : Subsystem  Description=|
      | 对原始转速做一阶低通，减小采样抖动
      | 
      | 每次把本拍输入与上次滤波结果按比例相加：
      | 本拍输出=α×本拍输入+β×上次输出；
      | α=Ts/(T+Ts)，β=T/(T+Ts)。
      | 
      | 当前T=0.067 s，Ts=Ts_ms/1000=0.02 s，因此α约0.229885、β约0.770115。新输入约占23%，旧结果约占77%。例如上次输出100、本次输入200，本次滤波结果约123，随后逐步靠近200。
      | 
      | 它抑制快速波动，也会让真实变化稍有滞后；不负责把ADC计数变成物理量，也不单凭滤波判定传感器故障。输出送Origin_Nc_Filter，供控制及记录链路使用。
      settings: AttributesFormatString=Origin_Nc_Filter（物理转速滤波）
  Subsystem2 : Subsystem  Description=|
      | 在滤波前检查排温是否超过930度
      | 
      | 输入来自Calibrating_T4，是已经标定成℃、但还没有低通滤波的排温。Constant1给出930 ℃上限，Xlim_Xdot_Judge负责判断与恢复确认，Unit Delay1保存上一有效温度。
      | 
      | 排温超过930 ℃时，图表置X_Flag_Locking，并把内部温度输出保持为上次有效值。恢复到上限内后不是立即清标志，而要经过连续确认，计数CNT_X大于5才解除。当前图表没有相邻温度变化率判断。
      | 
      | 本层只把故障标志Flag_T4_ExtreFailure送出；图表的X_Out仅反馈到记忆块，没有替换AnalogFilter_T4主温度路径。所以这不是“主排温被930限幅”的模块。
      | 
      | 该标志进入Sensor总线，但当前没有查到下游Bus Selector取用。它具备检测计算，不能因此认定它已接上自动停车。
      settings: AttributesFormatString=Subsystem2（子系统2）
  S_Sensor : Outport
      settings: AttributesFormatString=S_Sensor（传感器）
  wires:
  Bus Creator3/1 -> S_Sensor/1  "Sensor（传感器信息总线）"
  S_Nc/1 -> Data Type Conversion2/1
  S_T1t_calc/1 -> AnalogFilter_Nc/1(T1t_calc)
  S_SWI_Eblast/1 -> Bus Creator3/14  "SWI_Eblast（副油阀反馈）"
  S_SWI_EValve/1 -> Bus Creator3/13  "SWI_EValve（主油阀反馈）"
  S_SWI_Firework/1 -> Bus Creator3/12  "SWI_Firework（点火器告警反馈）"
  AnalogFilter_Nc/6(Ncr_Percent) -> Bus Creator3/10  "Ncr_Percent（归一化控制器转速百分比）"
  AnalogFilter_Nc/5(Ncr) -> Bus Creator3/9  "Ncr（归一化控制器转速）"
  AnalogFilter_Nc/4(Nc_Percent) -> Bus Creator3/8  "Nc_Percent（转速百分比）"
  AnalogFilter_Nc/3(Nc_Filter) -> Bus Creator3/7  "Nc_Filter（滤波后转速）"
  AnalogFilter_Nc/2(Ncdot_Flag_Locking) -> Bus Creator3/6  "Ncdot_Flag_Locking（转速变化率锁定标志）"
  AnalogFilter_Nc/1(Nc_Flag_Locking) -> Bus Creator3/5  "Nc_Flag_Locking（转速信号锁定标志）"
  Data Type Conversion2/1 -> AnalogFilter_Nc/2(S_Nc), Origin_Nc_Filter/1(In1)
  S_T4/1 -> Calibrating_T4/1(In1)
  Calibrating_T4/1(out) -> AnalogFilter_T4/1(In1), Subsystem2/1(In1)
  Calibrating_Tecu/1(out) -> Bus Creator3/4  "Tecu（处理器温度）"
  S_EngineState/1 -> AnalogFilter_Nc/3(S_EngineState)
  Origin_Nc_Filter/1(Out1) -> Bus Creator3/11, [Origin_Nc]  "Origin_Nc（原位转速）"
  S_SWI_ValveErr/1 -> Bus Creator3/15  "SWI_ValveErr（阀门综合告警反馈）"
  S_SWI_BleedAir/1 -> Bus Creator3/16  "SWI_BleedAir（引气阀反馈）"
  Subsystem2/1(Flag_T4_ExtreFailure) -> Bus Creator3/1  "Flag_T4_ExtreFailure（排温超限故障标志）"
  AnalogFilter_Poil/1(POil_Filter) -> Bus Creator3/17  "POil_Filter（滤波后燃油压力）"
  Calibrating_Poil/1(out) -> AnalogFilter_Poil/1(In1)
  S_Vpower/1 -> Bus Creator3/3  "Vpower（电源电压）"
  S_T0/1 -> Calibrating_T0/1(In1)
  Calibrating_T0/1(out) -> Bus Creator3/18, HuanSuanN/2(In2)  "T0（入口总温）"
  [Origin_Nc] -> HuanSuanN/1(In1)
  HuanSuanN/1(out) -> Bus Creator3/19  "HuanSuanZhuanSu（温度修正转速）"
  AnalogFilter_T4/1(T4_Filter) -> Bus Creator3/2  "T4_Filter（滤波后排气温度）"
  S_POil/1 -> Calibrating_Poil/1(In1)
  S_Tecu/1 -> Calibrating_Tecu/1(In1)

== system turbo_controller/COMMRead_ISM/MySet_Rxdatan_Read ==
  note: 从配置数据里取出软件版本的三个部分
      |
      | 按协议位置分别提取高、中、低版本字段，输出Soft_H、Soft_M、Soft_L。这里不做ADC采样、不比较
      | 版本新旧，也不把三个字段合成转速或压力。
      |
      | 这三项后续参与状态记录或回传，使上位机能识别当前控制软件版本。各字节的含义由配置协议约定；
      | 例如高、中、低分别是1、2、3时，它们仍是三个独立字段，并非自动成为十进制123。
  S_MySet_Rxdata : Inport
      settings: AttributesFormatString=S_MySet_Rxdata（板端配置缓冲区）
  BanBenHao_H : Selector  IndexMode=Zero-based  InputPortWidth=50  IndexOptions=Index vector (dialog)  Indices=[11]  OutputSizes=1
      settings: AttributesFormatString=BanBenHao_H（版本号高位）
  BanBenHao_L : Selector  IndexMode=Zero-based  InputPortWidth=50  IndexOptions=Index vector (dialog)  Indices=[13]  OutputSizes=1
      settings: AttributesFormatString=BanBenHao_L（版本号低位）
  BanBenHao_M : Selector  IndexMode=Zero-based  InputPortWidth=50  IndexOptions=Index vector (dialog)  Indices=[12]  OutputSizes=1
      settings: AttributesFormatString=BanBenHao_M（版本号中位）
  S_Soft_H : Outport
      settings: AttributesFormatString=S_Soft_H（软件版本高字节）
  S_Soft_M : Outport  Port=2
      settings: AttributesFormatString=S_Soft_M（软件版本中字节）
  S_Soft_L : Outport  Port=3
      settings: AttributesFormatString=S_Soft_L（软件版本低字节）
  wires:
  S_MySet_Rxdata/1 -> BanBenHao_L/1, BanBenHao_M/1, BanBenHao_H/1
  BanBenHao_H/1 -> S_Soft_H/1
  BanBenHao_M/1 -> S_Soft_M/1
  BanBenHao_L/1 -> S_Soft_L/1
